simulink model "FinalDesignObserverControl"  (R2024b)
settings: Solver=VariableStepAuto  StartTime=0.0  StopTime=tEnd  RelTol=1e-3
values from neighbouring files (symbols this model uses):
  A = [0       0    1     0 ... (first row only)    [FinalSettingsForObserverControl.m]
  B = [0       0 ... (first row only)    [FinalSettingsForObserverControl.m]
  Cm = [1 0 0 0 ... (first row only)    [FinalSettingsForObserverControl.m]
  dist_end_x = 700    [FinalSettingsForObserverControl.m]
  dist_end_y = 2000    [FinalSettingsForObserverControl.m]
  dist_Fx_x = 00    (= 0)    [FinalSettingsForObserverControl.m]
  dist_Fy = 0    [FinalSettingsForObserverControl.m]
  dist_start_x = 500    [FinalSettingsForObserverControl.m]
  dist_start_y = 0    [FinalSettingsForObserverControl.m]
  Fx_max = 400    [FinalSettingsForObserverControl.m]
  Fx_min = -Fx_max    (= -400)    [FinalSettingsForObserverControl.m]
  Fy_max = 400    [FinalSettingsForObserverControl.m]
  Fy_min = -Fy_max    (= -400)    [FinalSettingsForObserverControl.m]
  g_force = 1/mPlant    (= 8e-05)    [FinalSettingsForObserverControl.m]
  K = [kp + 3*mc*n^2,  0,    kd,       2*mc*n ... (first row only)    [FinalSettingsForObserverControl.m]
  Kix = mc*pI*wn^2    (= 0.459375)    [FinalSettingsForObserverControl.m]
  Kiy = Kix    (= 0.459375)    [FinalSettingsForObserverControl.m]
  L = place(A.', Cm.', p_obs).'    [FinalSettingsForObserverControl.m]
  mc = 12500    [FinalSettingsForObserverControl.m]
  n = sqrt(mu/r^3)    [FinalSettingsForObserverControl.m]
  r = 6.796e6    (= 6796000)    [FinalSettingsForObserverControl.m]
  useNonlinearPlant = true    [FinalSettingsForObserverControl.m]
  vx0 = 0    [FinalSettingsForObserverControl.m]
  vy0 = 0    [FinalSettingsForObserverControl.m]
  x0 = 100    [FinalSettingsForObserverControl.m]
  x_ref = 0    [FinalSettingsForObserverControl.m]
  y0 = 100    [FinalSettingsForObserverControl.m]
  y_ref = 0    [FinalSettingsForObserverControl.m]
  zhat0 = [xhat0; yhat0; vxhat0; vyhat0]    [FinalSettingsForObserverControl.m]
settings Model: Creator=USER  LastModifiedBy=USER

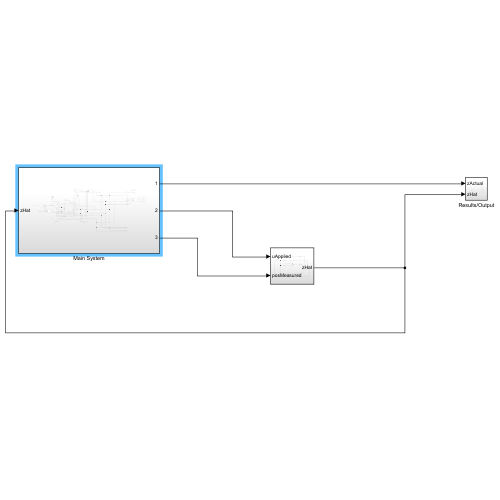
[thumbnail: Simulink's stored preview of the top-level diagram]
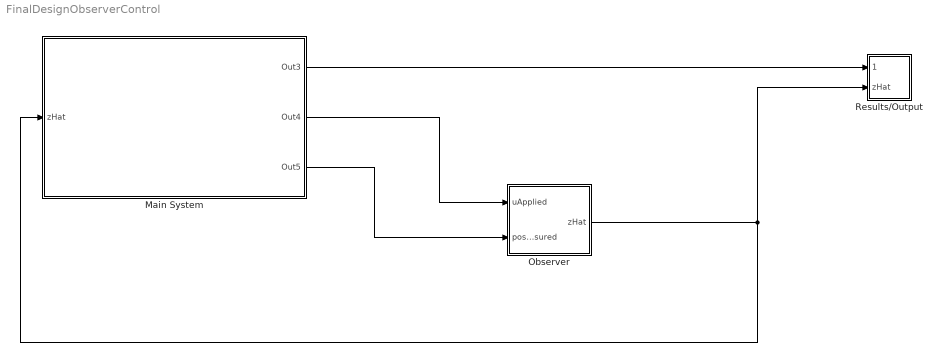
== system FinalDesignObserverControl ==
  Main System : Subsystem
  Observer : Subsystem
  Results/Output : Subsystem
  wires:
  Observer/1(zHat) -> Results/Output/2(zHat), Main System/1(zHat)
  Main System/1(Out3) -> Results/Output/1(zActual)
  Main System/2(Out4) -> Observer/1(uApplied)
  Main System/3(Out5) -> Observer/2(posMeasured)

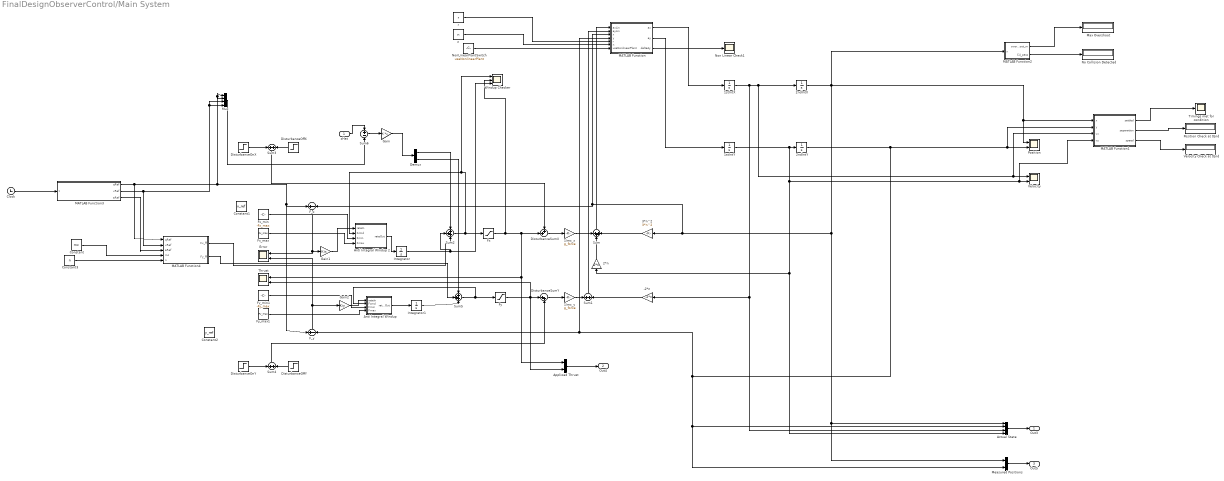
== system FinalDesignObserverControl/Main System ==
  zHat : Inport
  -2*n : Gain  Gain=-2*n
  1/mc_x : Gain  Gain=g_force
  1/mc_y : Gain  Gain=g_force
  1stIntX : Integrator  InitialCondition=vx0
  1stIntY : Integrator  InitialCondition=vy0
  2*n : Gain  Gain=2*n
  2ndIntX : Integrator  InitialCondition=x0
  2ndIntY : Integrator  InitialCondition=y0
  3*n^2 : Gain  Gain=3*n^2
  Actual State : Mux
  Anti Integral Windup : MATLAB Function  TreatAsAtomicUnit=on
  Anti Integral Windup 2 : MATLAB Function  TreatAsAtomicUnit=on
  Applioed Thrust : Mux  Inputs=2
  Clock : Clock
  Constant : Constant  Value=mc
  Constant1 : Constant  Value=x_ref
  Constant2 : Constant  Value=y_ref
  Constant3 : Constant  Value=n
  Demux : Demux  Outputs=2
  DisturbanceOffX : Step  Time=dist_end_x  After=-dist_Fx_x  SampleTime=0
  DisturbanceOffY : Step  Time=dist_end_y  After=-dist_Fy  SampleTime=0
  DisturbanceOnX : Step  Time=dist_start_x  After=dist_Fx_x  SampleTime=0
  DisturbanceOnY : Step  Time=dist_start_y  After=dist_Fy  SampleTime=0
  DisturbanceSumX : Sum  Inputs=++|
  DisturbanceSumY : Sum  Inputs=|++
  Error : Scope  NumInputPorts=2
  F_x : Sum  Inputs=+-
  F_y : Sum  Inputs=+-
  Fx : Saturate  UpperLimit=Fx_max  LowerLimit=Fx_min
  Fx_max : Constant  Value=Fx_max
  Fx_min : Constant  Value=-Fx_max
  Fy : Saturate  UpperLimit=Fy_max  LowerLimit=Fy_min
  Fy_max1 : Constant  Value=Fy_max
  Fy_min1 : Constant  Value=-Fy_max
  Gain : Gain  Gain=-K  Multiplication=Matrix(K*u)
  Gain1 : Gain  Gain=Kix
  Gain2 : Gain  Gain=Kiy
  Integrator : Integrator
  Integrator1 : Integrator
  MATLAB Function : MATLAB Function  TreatAsAtomicUnit=on
  MATLAB Function1 : MATLAB Function  TreatAsAtomicUnit=on
  MATLAB Function2 : MATLAB Function  TreatAsAtomicUnit=on
  MATLAB Function3 : MATLAB Function  TreatAsAtomicUnit=on
  MATLAB Function4 : MATLAB Function  TreatAsAtomicUnit=on
  Max Overshoot : Display
  Measured Positions : Mux  Inputs=2
  Mux : Mux
  No Collision Detected : Display
  Non Linear Check1 : Scope
  NonLinearPlantSwitch : Constant  Value=useNonlinearPlant
  Position : Scope  NumInputPorts=2
  Position Check at tEnd : Display
  Sum : Sum  Inputs=+++
  Sum1 : Sum  Inputs=+|+
  Sum2 : Sum  Inputs=+++
  Sum3 : Sum  Inputs=+|+
  Sum4 : Sum  Inputs=+|+
  Sum5 : Sum  Inputs=+++
  Sum6 : Sum  Inputs=+-
  Thrust : Scope  NumInputPorts=2
  Timings met for condition : Scope
  Velocity : Scope  NumInputPorts=2
  Velocity Check at tEnd : Display
  Windup Checker : Scope  NumInputPorts=3
  n : Constant  Value=n
  r : Constant  Value=r
  Out3 : Outport
  Out4 : Outport  Port=2
  Out5 : Outport  Port=3
  wires:
  1stIntY/1 -> 2ndIntY/1, Actual State/4, 2*n/1, MATLAB Function1/4(vy), Velocity/2
  F_y/1 -> Gain2/1, Error/2
  DisturbanceSumX/1 -> 1/mc_x/1
  2ndIntY/1 -> MATLAB Function1/2(y), Position/2, Measured Positions/2, Actual State/2, F_y/2, MATLAB Function/4(y)
  Actual State/1 -> Out3/1
  r/1 -> MATLAB Function/5(r)
  Measured Positions/1 -> Out5/1
  DisturbanceOnY/1 -> Sum4/1
  DisturbanceSumY/1 -> 1/mc_y/1
  n/1 -> MATLAB Function/6(n)
  MATLAB Function/1(ax) -> 1stIntX/1
  F_x/1 -> Gain1/1, Error/1
  DisturbanceOffY/1 -> Sum4/2
  DisturbanceOffX/1 -> Sum3/2
  MATLAB Function/2(ay) -> 1stIntY/1
  DisturbanceOnX/1 -> Sum3/1
  Sum1/1 -> MATLAB Function/2(ayLin)
  Sum/1 -> MATLAB Function/1(axLin)
  NonLinearPlantSwitch/1 -> MATLAB Function/7(useNonlinearPlant)
  MATLAB Function/3(deltaAy) -> Non Linear Check1/1
  Applioed Thrust/1 -> Out4/1
  Sum3/1 -> DisturbanceSumX/1
  1stIntX/1 -> Actual State/3, -2*n/1, MATLAB Function1/3(vx), Velocity/1, 2ndIntX/1
  3*n^2/1 -> Sum/3
  1/mc_x/1 -> Sum/1
  2*n/1 -> Sum/2
  1/mc_y/1 -> Sum1/1
  -2*n/1 -> Sum1/2
  Gain/1 -> Demux/1
  Demux/2 -> Sum5/1
  Fy/1 -> Applioed Thrust/2, Thrust/2, DisturbanceSumY/1
  Sum2/1 -> Windup Checker/1, Anti Integral Windup 2/2(Fcmd), Fx/1
  Sum5/1 -> Anti Integral Windup/2(Fcmd), Fy/1
  Demux/1 -> Sum2/1
  Sum4/1 -> DisturbanceSumY/2
  Integrator/1 -> Windup Checker/3, Sum2/2
  Fx/1 -> Windup Checker/2, DisturbanceSumX/2, Thrust/1, Applioed Thrust/1
  2ndIntX/1 -> MATLAB Function2/1(x), F_x/2, MATLAB Function/3(x), 3*n^2/1, Measured Positions/1, Actual State/1, Position/1, MATLAB Function1/1(x)
  MATLAB Function1/1(settled) -> Timings met for condition/1
  MATLAB Function1/2(separation) -> Position Check at tEnd/1
  MATLAB Function1/3(speed) -> Velocity Check at tEnd/1
  Gain1/1 -> Anti Integral Windup 2/1(rateIn)
  Anti Integral Windup 2/1(rateOut) -> Integrator/1
  Fx_max/1 -> Anti Integral Windup 2/4(Fmax)
  Fx_min/1 -> Anti Integral Windup 2/3(Fmin)
  Gain2/1 -> Anti Integral Windup/1(rateIn)
  Fy_min1/1 -> Anti Integral Windup/3(Fmin)
  Fy_max1/1 -> Anti Integral Windup/4(Fmax)
  Anti Integral Windup/1(rateOut) -> Integrator1/1
  MATLAB Function2/1(overshoot_m) -> Max Overshoot/1
  MATLAB Function2/2(C4_pass) -> No Collision Detected/1
  Clock/1 -> MATLAB Function3/1(t)
  MATLAB Function3/1(qRef) -> MATLAB Function4/1(qRef), Mux/1, Mux/2, F_x/1, F_y/1
  MATLAB Function3/2(vRef) -> MATLAB Function4/2(vRef), Mux/3, Mux/4
  Mux/1 -> Sum6/2
  zHat/1 -> Sum6/1
  Sum6/1 -> Gain/1
  MATLAB Function3/3(aRef) -> MATLAB Function4/3(aRef)
  Constant/1 -> MATLAB Function4/4(mc)
  Constant3/1 -> MATLAB Function4/5(n)
  MATLAB Function4/1(Fx_ff) -> Sum2/3
  MATLAB Function4/2(Fy_ff) -> Sum5/2
  Integrator1/1 -> Sum5/3

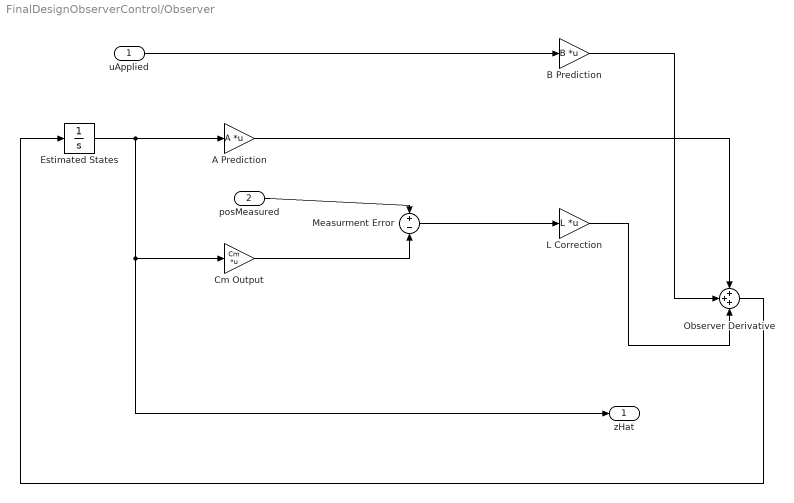
== system FinalDesignObserverControl/Observer ==
  uApplied : Inport
  posMeasured : Inport  Port=2
  A Prediction : Gain  Gain=A  Multiplication=Matrix(K*u)
  B Prediction : Gain  Gain=B  Multiplication=Matrix(K*u)
  Cm Output : Gain  Gain=Cm  Multiplication=Matrix(K*u)
  Estimated States : Integrator  InitialCondition=zhat0
  L Correction : Gain  Gain=L  Multiplication=Matrix(K*u)
  Measurment Error : Sum  Inputs=+-
  Observer Derivative : Sum  Inputs=+++
  zHat : Outport
  wires:
  L Correction/1 -> Observer Derivative/3
  Cm Output/1 -> Measurment Error/2
  posMeasured/1 -> Measurment Error/1
  A Prediction/1 -> Observer Derivative/1
  Estimated States/1 -> zHat/1, Cm Output/1, A Prediction/1
  Observer Derivative/1 -> Estimated States/1
  Measurment Error/1 -> L Correction/1
  B Prediction/1 -> Observer Derivative/2
  uApplied/1 -> B Prediction/1

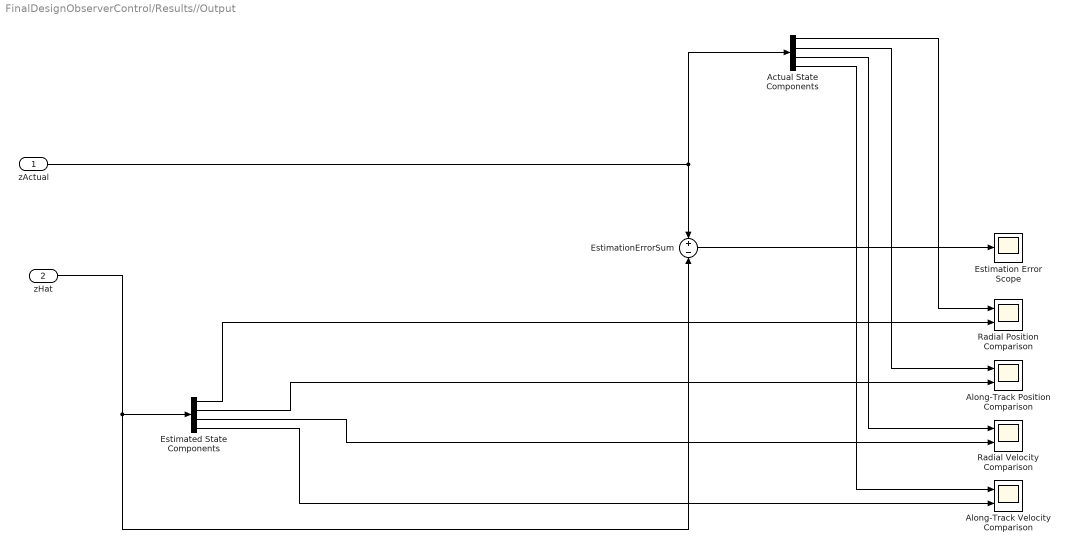
== system FinalDesignObserverControl/Results//Output ==
  zActual : Inport
  zHat : Inport  Port=2
  Actual State Components : Demux
  Along-Track Position Comparison : Scope  NumInputPorts=2
  Along-Track Velocity Comparison : Scope  NumInputPorts=2
  Estimated State Components : Demux
  Estimation Error Scope : Scope
  EstimationErrorSum : Sum  Inputs=+-
  Radial Position Comparison : Scope  NumInputPorts=2
  Radial Velocity Comparison : Scope  NumInputPorts=2
  wires:
  Estimated State Components/4 -> Along-Track Velocity Comparison/2
  zHat/1 -> EstimationErrorSum/2, Estimated State Components/1
  EstimationErrorSum/1 -> Estimation Error Scope/1
  Estimated State Components/2 -> Along-Track Position Comparison/2
  Estimated State Components/3 -> Radial Velocity Comparison/2
  Actual State Components/2 -> Along-Track Position Comparison/1
  Estimated State Components/1 -> Radial Position Comparison/2
  Actual State Components/3 -> Radial Velocity Comparison/1
  Actual State Components/1 -> Radial Position Comparison/1
  zActual/1 -> EstimationErrorSum/1, Actual State Components/1
  Actual State Components/4 -> Along-Track Velocity Comparison/1

== matlab function FinalDesignObserverControl/Main System/MATLAB Function1 ==
  data: x input; y input; vx input; settled output; vy input; separation output; speed output
function [settled, separation, speed] = checkDocking(x, y, vx, vy)
separation = hypot(x, y);       % metres from target
speed      = hypot(vx, vy);     % relative speed in m/s
settled    = (separation <= 0.10) && (speed <= 0.01);
end

== matlab function FinalDesignObserverControl/Main System/MATLAB Function ==
  data: axLin input; ax output; ayLin input; x input; y input; r input; n input; useNonlinearPlant input; ay output; deltaAy output
function [ax, ay, deltaAy] = selectPlant(axLin, ayLin, x, y, r, n, useNonlinearPlant)

% Linear mode: pass the existing accelerations straight through.
ax = axLin;
ay = ayLin;
deltaAy = 0;

if useNonlinearPlant
    rc = hypot(r + x, y);                     % Chaser distance from Earth [m]
    dr = (2*r*x + x*x + y*y) / (rc + r);    % Equivalent to rc - r [m]

    % Gravity coefficient: g = n^2 - mu/rc^3, using mu = n^2*r^3
    g = n^2 * (dr/rc) * (1 + r/rc + (r/rc)^2);

    deltaAy = y*g;                            % Along-track correction [m/s^2]
    ax = axLin + ((r + x)*g - 3*n^2*x);
    ay = ayLin + deltaAy;
end
end

== matlab function FinalDesignObserverControl/Main System/Anti Integral Windup 2 ==
  data: rateIn input; rateOut output; Fcmd input; Fmin input; Fmax input
function rateOut = antiWindup(rateIn, Fcmd, Fmin, Fmax)
% rateIn is Ki * position error, in N/s.
if (Fcmd >= Fmax && rateIn > 0) || (Fcmd <= Fmin && rateIn < 0)
    rateOut = 0;
else
    rateOut = rateIn;
end
end

== matlab function FinalDesignObserverControl/Main System/Anti Integral Windup ==
  data: rateIn input; rateOut output; Fcmd input; Fmin input; Fmax input
function rateOut = antiWindup(rateIn, Fcmd, Fmin, Fmax)
% rateIn is Ki * position error, in N/s.
if (Fcmd >= Fmax && rateIn > 0) || (Fcmd <= Fmin && rateIn < 0)
    rateOut = 0;
else
    rateOut = rateIn;
end
end

== matlab function FinalDesignObserverControl/Main System/MATLAB Function2 ==
  settings: updateMethod=DISCRETE  sampleTime=0.01
  data: x input; overshoot_m output; C4_pass output
function [overshoot_m, C4_pass] = checkC4(x)
% Track the greatest distance travelled past the docking port [m].
persistent maxOvershoot

if isempty(maxOvershoot)
    maxOvershoot = 0;
end

maxOvershoot = max(maxOvershoot, -x);
overshoot_m = maxOvershoot;
C4_pass = (overshoot_m <= 0.10);
end

== matlab function FinalDesignObserverControl/Main System/MATLAB Function3 ==
  data: t input; qRef output; vRef output; aRef output
function [qRef, vRef, aRef] = approachReference(t)
T = 350;                         % Approach duration [s]
u = min(max(t/T, 0), 1);

qRef = 100*(1 - 10*u^3 + 15*u^4 - 6*u^5);       % [m]
vRef = (100/T)*(-30*u^2 + 60*u^3 - 30*u^4);     % [m/s]
aRef = (100/T^2)*(-60*u + 180*u^2 - 120*u^3);   % [m/s^2]
end

== matlab function FinalDesignObserverControl/Main System/MATLAB Function4 ==
  data: qRef input; Fx_ff output; vRef input; aRef input; mc input; n input; Fy_ff output
function [Fx_ff, Fy_ff] = thrustFeedforward(qRef, vRef, aRef, mc, n)
Fx_ff = mc*(aRef - 3*n^2*qRef - 2*n*vRef);
Fy_ff = mc*(aRef + 2*n*vRef);
end
